simulink model "tDoubleActingPistonCylinder"  (R2025b)
settings: Solver=VariableStepAuto  StartTime=0.0  StopTime=10.0  RelTol=1e-3
libraries: fl_lib x3, customization_lib x3, nesl_utility x1
settings Model: Creator=ndegoede  LastModifiedBy=ndegoede
settings SimscapeCC: SimscapeLogType=all  SimscapeLogOpenViewer=on

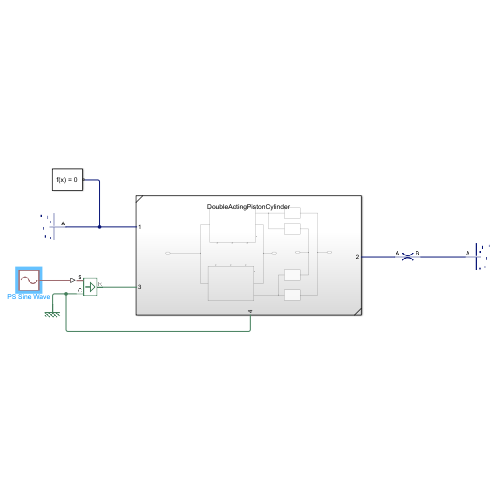
[thumbnail: Simulink's stored preview of the top-level diagram]
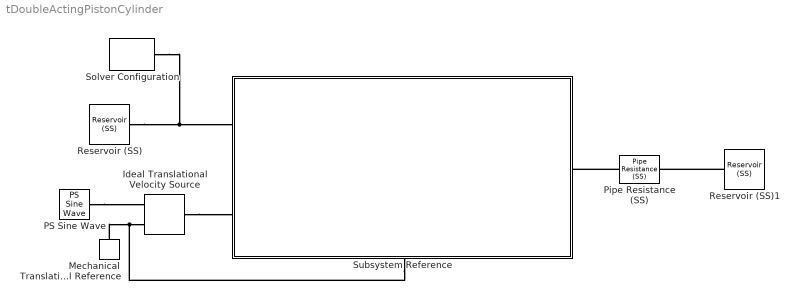
== system tDoubleActingPistonCylinder ==
  Ideal Translational Velocity Source : fl_lib/Mechanical/Mechanical Sources/Ideal Translational Velocity Source
  Mechanical Translational Reference : fl_lib/Mechanical/Translational Elements/Mechanical Translational Reference
  PS Sine Wave : fl_lib/Physical Signals/Sources/PS Sine Wave  amplitude=20 cm/s  bias=0  frequency_spec=foundation.enum.frequencySpec.frequencySI  frequency_SI=1 Hz  frequency_angular=1 rad/s  phase=pi/4 rad
      settings: InternalSimscapePortConfiguration="{\"Bottom\":[],\"Left\":[],\"Right\":[{\"id\":\"O\",\"label\":\"\",\"type\":\"output\"}],\"Top\":[]}"
  Pipe Resistance (SS) : customization_lib/solution/elements/Pipe Resistance (SS)  length=5 m  area=0.01 m^2  Dh=0.1128 m  roughness=15e-6 m  Re_lam=2000  Re_tur=4000  shape_factor=64  custom_ports=false  length_A=1e-3 m  length_B=1e-3 m
      settings: SourceProductName=Customization  InternalSimscapePortConfiguration="{\"Bottom\":[],\"Left\":[{\"id\":\"A\",\"label\":\"A\",\"type\":\"customization.solution.solution\"}],\"Right\":[{\"id\":\"B\",\"label\":\"B\",\"type\":\"customization.solution.solution\"}],\"Top\":[]}"
  Reservoir (SS) : customization_lib/solution/elements/Reservoir (SS)  pressure_spec=foundation.enum.pressure_spec.specified  reservoir_pressure=1 MPa  reservoir_temperature=293.15 K  reservoir_concentration=0 kg/m^3  area=0.01 m^2  custom_ports=false  length_A=1e-3 m
      settings: SourceProductName=Customization  InternalSimscapePortConfiguration="{\"Bottom\":[],\"Left\":[{\"id\":\"A\",\"label\":\"A\",\"type\":\"customization.solution.solution\"}],\"Right\":[],\"Top\":[]}"
  Reservoir (SS)1 : customization_lib/solution/elements/Reservoir (SS)  pressure_spec=foundation.enum.pressure_spec.specified  reservoir_pressure=3 MPa  reservoir_temperature=293.15 K  reservoir_concentration=0 kg/m^3  area=0.01 m^2  custom_ports=false  length_A=1e-3 m
      settings: SourceProductName=Customization  InternalSimscapePortConfiguration="{\"Bottom\":[],\"Left\":[{\"id\":\"A\",\"label\":\"A\",\"type\":\"customization.solution.solution\"}],\"Right\":[],\"Top\":[]}"
  Solver Configuration : nesl_utility/Solver Configuration  PhysicalDomain=network_engine_domain  SubClassName=solver  LeftPortType=input  RightPortType=generic  Tones=[]  Harmonics=[]  SimulateNoise=off  Profile=off  UseLocalSampling=off  EnableSwitchedLinearOptims=on  FrequencyDomain=off  UseCCode=off  RelTol=0.001  AbsTol=0.001  MinStep=1e-09  ToWorkspace=off  RevertToSquareIcSolve=off  NumHomotopyIterations=100  PhasorMode=off  PhasorModeNumHarmonics=1  ConsistencySolver=NEWTON_XTOL_AFTER_FTOL  IndexReductionMethod=DerivativeReplacement  DoDC=off  ResidualTolerance=1e-09  ConsistencyTolSource=GLOBAL  ConsistencyAbsTol=0.001  ConsistencyRelTol=0.001  ConsistencyTolFactor=0.001  UseLocalSolver=off  LocalSolverChoice=NE_BACKWARD_EULER_ADVANCER  ResolveIndetEquations=on  FunctionEvalNumThread=1  LocalSolverSampleTime=0.001  DoFixedCost=off  MaxNonlinIter=3  MaxModeIter=2  ComputeImpulses=off  ImpulseIterations=2  LinearAlgebra=auto  LinearAlgebraNumThread=0  EquationFormulation=NE_TIME_EF  DelaysMemoryBudget=1024  AutomaticFiltering=on  FilteringTimeConstant=0.001  PartitionStorageMethod=AS_NEEDED  PartitionMemoryBudget=1024  PartitionMethod=ROBUST  MultibodyUseLocalSolver=off  MultibodyLocalSolverChoice=ODE1  MultibodyLocalSolverSampleTime=0.001
  Subsystem Reference : Subsystem  ReferencedSubsystem=DoubleActingPistonCylinder
      settings: PortSchema="{\"entries\":[{\"content\":{\"sides\":[{\"content\":{\"connectorIds\":[\"LConn1\",\"LConn3\"]},\"type\":\"ConnectorPlacement.EquallySpacedRectSide\",\"uuid\":\"8acd0945-963f-4ac9-9e22-6ebef24fa469\"},{\"content\":{\"connectorIds\":[\"LConn2\"],\"side\":\"RIGHT\"},\"type\":\"ConnectorPlacement.EquallySpacedRectSide\",\"uuid\":\"3b4a74cd-deb1-4dcf-bacc-c9108daeb4d0\"},{\"content\":{\"side\":\"TOP\"},\"type\":\"ConnectorPlacement.EquallySpacedRectSide\",\"uuid\":\"b26b8698-1eb6-4b70-b966-bc7275cbd4a0\"},{\"content\":{\"connectorIds\":[\"LConn4\"],\"side\":\"BOTTOM\"},\"type\":\"ConnectorPlacement.EquallySpacedRectSide\",\"uuid\":\"df97d8fb-7bd4-42c8-81cb-d93f7329400b\"}]},\"type\":\"ConnectorPlacement.EquallySpacedConnector\",\"uuid\":\"8ea66071-78df-4809-a2e0-9adf4b1871fd\"}],\"packageUris\":[\"http://schema.mathworks.com/mf0/Connector/R2020b\"],\"version\":\"1.0\"}"
  connections:
  Reservoir (SS)/LConn1 -- Solver Configuration/RConn1 -- Subsystem Reference/LConn1
  Pipe Resistance (SS)/LConn1 -- Subsystem Reference/LConn2
  Reservoir (SS)1/LConn1 -- Pipe Resistance (SS)/RConn1
  Ideal Translational Velocity Source/LConn1 -- Subsystem Reference/LConn3
  Mechanical Translational Reference/LConn1 -- Subsystem Reference/LConn4 -- Ideal Translational Velocity Source/RConn2
  PS Sine Wave/RConn1 -- Ideal Translational Velocity Source/RConn1
